simulink model "ball_impact"  (Simulink 8.1)
settings: Solver=ode4  SolverMode=SingleTasking  StartTime=0.0  StopTime=inf  FixedStep=0.0005  RelTol=1e-3
StartFcn:
  |  warndlg('Dexterit-E models cannot run under simulation. Please compile your model and run it from within Dexterit-E.');set_param(bdroot,'SimulationCommand','stop')
undefined symbols (not defined in the file or in its folder): CreateParameterTableGUI, slselsubs
libraries: xpclib x30, simulink x8, KINARM_general x3, KINARM_loads x2, Video x2, KINARM_EP_loads x1
(part 4 of 5)

== matlab function DataLogging/Poll KINARM/Create KINARM Data Array ==
  settings: fimath=|
      | fimath(...
      | 'RoundMode', 'floor',...
      | 'OverflowMode', 'wrap',...
      | 'ProductMode', 'KeepLSB', 'ProductWordLength', 32,...
      | 'SumMode', 'KeepLSB', 'SumWordLength', 32,...
      | 'CastBeforeSum', false)
  data: robot_calibrations input double; robot_hardware_settings input double; force_sensor_data input double; robot_data input double; servo_update_count input double; delay_estimates input double; primary_encoder_data input double; ep_calibration_button_bitfield input double; torque_command input double; hand_feedback_settings input double; kinarm_data output double; dominant_arm input double; primary_encoder_data_out output double; gaze_data input double
% This function constructs a matrix of KINARM-related data called "KINdata". This matrix consists of three rows: the first two are each
% for data related to the respective robot (i.e. row 1 is for robot 1 data, row 2 for robot 2 data, etc.), and the third row is for data
% not specific to either arm. Each row of the matrix is currently of length 50, though not all elements in each row are used.
function [kinarm_data, primary_encoder_data_out]= create_KINARM_data_array(robot_calibrations, robot_hardware_settings, force_sensor_data, ...
                                                      robot_data, servo_update_count, delay_estimates, primary_encoder_data, ...
                                                      ep_calibration_button_bitfield, torque_command, hand_feedback_settings, dominant_arm, gaze_data)

kinarm_data = zeros(3,50);
primary_encoder_data_out = zeros(2,6);

% Create the rows of robot-specific data. The utility function create_robot_row is used to assemble the values for each row. 
% The last section of that function (in which the row elements are assigned individually) documents the row contents.
kinarm_data(1,:) = create_robot_row(robot_calibrations(1:8), robot_hardware_settings(1:12), ...
                                    force_sensor_data(1:7), robot_data(1:10), torque_command(1:2));

kinarm_data(2,:) = create_robot_row(robot_calibrations(9:16), robot_hardware_settings(13:24), ...
                                    force_sensor_data(8:14), robot_data(11:20), torque_command(3:4));
								
% Create the last row of KINdata, which contains information not specific to any single arm.
kinarm_data(3,1) = dominant_arm;                     % dominant KINARM for the experiment (1: arm 1, 2: arm 2)
kinarm_data(3,2) = hand_feedback_settings(5);        % duration of feed forward for position of hand feedback (s)
kinarm_data(3,3) = hand_feedback_settings(1);        % hand feedback arm (0: none, 1: dominant, 2: non-dominant, 3: both, 4: controlled by task program)
kinarm_data(3,4) = hand_feedback_settings(2);        % hand feedback settings source (0: GUI, 1: from task program)
kinarm_data(3,5) = hand_feedback_settings(4);        % feedback colour (RRRGGGBBB string converted to integer)
kinarm_data(3,6) = hand_feedback_settings(3);        % feedback radius (m)
kinarm_data(3,7) = 1;                                % global load enable set by BKIN client software (no longer an option; thus always on)
kinarm_data(3,8) = delay_estimates(1);               % primary encoders velocity delay estimate (s)
kinarm_data(3,9) = delay_estimates(2);               % primary encoders acceleration delay estimate (s)
kinarm_data(3,10) = delay_estimates(3);              % secondary encoders velocity delay estimate (s)
kinarm_data(3,11) = delay_estimates(4);              % secondary encoders acceleration delay estimate (s)
kinarm_data(3,12) = servo_update_count;              % servo update count
kinarm_data(3,13) = ep_calibration_button_bitfield;  % EP calibration button status bitfield

gaze_available = gaze_data(1);
kinarm_data(3,14) = gaze_available;              % is Gaze tracking hardware available
kinarm_data(3,15) = hand_feedback_settings(6);   % Gaze feedback (0: on, 1: controlled by task program)

if gaze_available
    kinarm_data(3,16) = gaze_data(2);            % Gaze X location in global coordinates
    kinarm_data(3,17) = gaze_data(3);            % Gaze Y location in global coordinates
    kinarm_data(3,18) = gaze_data(4);            % Gaze Timestamp in seconds
    kinarm_data(3,19) = gaze_data(5);            % Gaze pupil area
    kinarm_data(3,20) = gaze_data(6);          % Gaze Event ID
    kinarm_data(3,21) = gaze_data(7);          % Gaze Event start time in seconds
    kinarm_data(3,22) = gaze_data(8);          % Gaze Event end time in seconds    
else
    kinarm_data(3,16) = -100;                    % Gaze X location in global coordinates
    kinarm_data(3,17) = -100;                    % Gaze Y location in global coordinates
    kinarm_data(3,18) = -100;                    % Gaze Timestamp in seconds
    kinarm_data(3,19) = -100;                    % Gaze Timestamp in seconds
end

% Create the two rows of primary encoder data. These outputs are analogous to the L1/L2 outputs in kinarm_data, the difference being that
% these are always derived from the primary encoders while the contents of kinarm_data is derived from the primary or secondary encoders
% (depending on the user's choice of whether or not to use the secondary encoders in the GUI).
for i = 1:2
	offset = (i-1)*6;
    
    relative_shoulder_angle = primary_encoder_data(1 + offset);
    relative_elbow_angle = primary_encoder_data(2 + offset);
    shoulder_velocity = primary_encoder_data(3 + offset);
    elbow_velocity = primary_encoder_data(4 + offset);
    shoulder_acceleration = primary_encoder_data(5 + offset);
    elbow_acceleration = primary_encoder_data(6 + offset);

    shoulder_angle_offset = robot_calibrations(1 + (i-1)*8);
    elbow_angle_offset = robot_calibrations(2 + (i-1)*8);
	L1 = robot_calibrations(5 + (i-1)*8);                               % L1 (upper arm segment) length (m)
	L3_error = robot_calibrations(8 + (i-1)*8);                         % L3 error, the difference between lengths L3 and L5 (m)
    
    hwoffset = (i-1)*12;
	robot_orientation = robot_hardware_settings(7 + hwoffset);          % robot orientation (1: right-handed from robot perspective, -1: left-handed from robot perspective)
 	L5 = robot_hardware_settings(3 + hwoffset);                         % L5 segment length (m)
	L2_L5_angle = robot_hardware_settings(4 + hwoffset);                % angle of L2 relative to L5 (rad)
    robot_type = robot_hardware_settings(1 + hwoffset);
    isExo = robot_type == 0 || robot_type == 2;
    
	% Before proceeding, the shoulder and elbow angles are shifted by the offsets determined by the calibration. If the calibration has been
	% performed correctly, this ensures that the angle of 0 corresponds to when the arm is aligned with the coronal plane. In the case of the 
	% elbow angle for a KINARM EXO, an extra correction is performed (using a utility function, and according to the current calibration) to 
	% account for small imperfections in the parallelogram of KINARM links caused by differences in the lengths of L3 and L5 (which are 
	% theoretically equal).
	shoulder_angle = relative_shoulder_angle + shoulder_angle_offset;

	% If the robot is an Exoskeleton, use the correct_elbow_angle function to account for imperfections on the KINARM robot parallelogram structure
	if isExo  
		[angle_corr, vel_corr, acc_corr] = correct_elbow_angle(relative_elbow_angle + elbow_angle_offset, elbow_velocity, elbow_acceleration, L2_L5_angle, L1, L5, L3_error);				
		elbow_angle = relative_elbow_angle + elbow_angle_offset + angle_corr;
		elbow_velocity = elbow_velocity + vel_corr;
		elbow_acceleration = elbow_acceleration + acc_corr;		
	else
		elbow_angle = relative_elbow_angle + elbow_angle_offset;
	end

    L1_angle = shoulder_angle;
    L2_angle = shoulder_angle + elbow_angle;

    L1_velocity = shoulder_velocity;
    L2_velocity = shoulder_velocity + elbow_velocity;

    L1_acceleration = shoulder_acceleration;
    L2_acceleration = shoulder_acceleration + elbow_acceleration;

	% a robot_orientation < 0 means that the robot is left-handed from its perspective (i.e. if you look at the robot structure, 
	% and pretend that it is a humanoid, the robot itself looks left-handed).  For an Exoskeleton robot, this is the
	% robot that the left-hand of the subject grabs. For an EP robot, this is the robot that the subjec'ts right-hand grabs.  
	
    if robot_orientation < 0
        L1_angle = -L1_angle + pi;
        L2_angle = -L2_angle + pi;

        L1_velocity = -L1_velocity;
        L2_velocity = -L2_velocity;

        L1_acceleration = -L1_acceleration;
        L2_acceleration = -L2_acceleration;
    end

    primary_encoder_data_out(i,1) = L1_angle;
    primary_encoder_data_out(i,2) = L2_angle;
    
    primary_encoder_data_out(i,3) = L1_velocity;
    primary_encoder_data_out(i,4) = L2_velocity;
    
    primary_encoder_data_out(i,5) = L1_acceleration;
    primary_encoder_data_out(i,6) = L2_acceleration;
end


%%%%%%%%%%%%%%%%%%%%%%%%%%%%%%%%%%%%%%%%%%%%%%%%%%%%%%%%%%%%%%%%%%%%%%%%%%%%%%%%%%%%%%%%%%%%%%%%%%%%%%%%%%%%%%%%%%%%%%%%
%%%%%%%%%%%%%%%%%%%%%%%%%%%%%%%%%%%%%%%%%%%%%%%%%%%%%%%%%%%%%%%%%%%%%%%%%%%%%%%%%%%%%%%%%%%%%%%%%%%%%%%%%%%%%%%%%%%%%%%%
% This function creates a row of arm-specific data for the KINARM data matrix. 
function robot_row = create_robot_row(calibration, hardware_settings, force_sensor_data, robot_data, torque_command)

% Extract the relevant information from each input array.
shoulder_angle_offset = calibration(1);            % offset added to motion control card shoulder angle to get real angle (rad)
elbow_angle_offset = calibration(2);               % offset added to motion control card elbow angle to get real angle (rad)
shoulder_position_x = calibration(3);              % shoulder x position (m) (global coordinates)
shoulder_position_y = calibration(4);              % shoulder y position (m) (global coordinates)
L1 = calibration(5);                               % L1 (upper arm segment) length (m)
L2 = calibration(6);                               % L2 (forearm segment) length (m); segment length puts distal end in line with subject pointer
pointer_offset = calibration(7);                   % perpendicular distance from L2 to subject pointer (m)
L3_error = calibration(8);                         % L3 error, the difference between lengths L3 and L5 (m)

robot_type = hardware_settings(1);                 % robot type (0: EXO, 1: EP, 2:NHP)
isExo = robot_type == 0 || robot_type == 2;
isEP = robot_type == 1;
L5 = hardware_settings(3);                         % L5 segment length (m)
L2_L5_angle = hardware_settings(4);                % angle of L2 relative to L5 (rad)
force_sensor_angle_offset = hardware_settings(5);  % offset of force sensor from forearm linkage (rad)
robot_orientation = hardware_settings(7);          % robot orientation (1: right-handed from robot perspective, -1: left-handed from robot perspective)

force_sensor_force_u = force_sensor_data(1);       % force sensor u force (N)
force_sensor_force_v = force_sensor_data(2);       % force sensor v force (N)
force_sensor_force_w = force_sensor_data(3);       % force sensor w force (N)
force_sensor_torque_u = force_sensor_data(4);      % force sensor u torque (Nm) 
force_sensor_torque_v = force_sensor_data(5);      % force sensor v torque (Nm)
force_sensor_torque_w = force_sensor_data(6);      % force sensor w torque (Nm)
force_sensor_timestamp = force_sensor_data(7);      % force sensor w torque (Nm)

relative_shoulder_angle = robot_data(1);        % current shoulder joint angle (rad)
relative_elbow_angle = robot_data(2);           % current elbow joint angle (rad)
shoulder_velocity = robot_data(3);                 % shoulder joint angular velocity (rad/s)
elbow_velocity = robot_data(4);                    % elbow joint angular velocity (rad/s)
shoulder_acceleration = robot_data(5);             % shoulder joint angular acceleration (rad/s^2)
elbow_acceleration = robot_data(6);                % elbow joint angular acceleration (rad/s^2)
filtered_shoulder_velocity = robot_data(7);        % filtered shoulder velocity (rad/s)
filtered_elbow_velocity = robot_data(8);           % filtered elbow velocity (rad/s)
motor1_status = robot_data(9);                     % motor 1 status
motor2_status = robot_data(10);                    % motor 2 status

shoulder_torque_cmd = torque_command(1);	       % commanded shoulder torque (Nm)
elbow_torque_cmd = torque_command(2);              % commanded elbow torque (Nm)



% With the inputs unpacked, start using them to compute other values that will be included in the data array. Some inputs are included in the
% array directly, but the kinematic data is also developed from the joint-based information supplied by the polling function into information 
% about the arm segments, the elbow, and the hand/fingertip as described in the following sections.

% Before proceeding, the shoulder and elbow angles are shifted by the offsets determined by the calibration. If the calibration has been
% performed correctly, this ensures that the angle of 0 corresponds to when the arm is aligned with the coronal plane. In the case of the 
% elbow angle for a KINARM EXO, an extra correction is performed (using a utility function, and according to the current calibration) to 
% account for small imperfections in the parallelogram of KINARM links caused by differences in the lengths of L3 and L5 (which are 
% theoretically equal).
shoulder_angle = relative_shoulder_angle + shoulder_angle_offset;

% If the robot is an Exoskeleton, use the correct_elbow_angle function to account for imperfections on the KINARM robot parallelogram structure
if isExo
	[angle_corr, vel_corr, acc_corr] = correct_elbow_angle(relative_elbow_angle + elbow_angle_offset, elbow_velocity, elbow_acceleration, L2_L5_angle, L1, L5, L3_error);
	elbow_angle = relative_elbow_angle + elbow_angle_offset + angle_corr;
	elbow_velocity = elbow_velocity + vel_corr;
	elbow_acceleration = elbow_acceleration + acc_corr;
else
	elbow_angle = relative_elbow_angle + elbow_angle_offset;
end

% Convert robot orientation as supplied in the hardware settings (a scaling factor used to calculate robot data) to the number 1 or 2,
% indicating which of the subject's arms will normally be using the robot: right or left, respectively. This is done to be consistent 
% with previous versions of the TDK. Note that the robot orientations of KINARM EP robots are "opposite" those for KINARM EXOs when.
if (isEP && robot_orientation < 0.0) || (isExo && robot_orientation > 0.0)
    arm_orientation = 1;  % right arm orientation expected for subject
else
    arm_orientation = 2;  % left arm orientation expected for subject
end

% Create a motor status variable for the robot that is consistent with previous versions of the TDK: the value forms a bitfield in
% which non-zero bits indicate a motor is disabled or faulted. The least significant bit is motor 1; the next is motor 2.
motor_status = motor2_status * 2 + motor1_status;

% Calculate segment information, i.e. positions, velocities, and accelerations for L1 and L2. "Segment-based" values here differ from the
% "joint-based" values in a few ways, though they are still expressed in angles:
%   i) elbow angles are no longer shoulder-relative (that is, L2 angles are not relative to L1)
%  ii) positions are expressed with the corrections calculated above
% iii) all angles are expressed in the same system, where 0 is the angular position of the exoskeleton right arm when aligned with the 
%      coronal plane and positive changes in angle correspond to counterclockwise movements.
%
% This section also determines the torque commands for motor 1 (shoulder) and motor 2 (elbow). When a positive torque is applied to the 
% forearm linkage by motor 2 it causes the same positive force on the upper arm linkage, so the torque applied to motor 1 is the desired
% shoulder torque less any torque commanded at the elbow.

L1_angle = shoulder_angle;
L2_angle = shoulder_angle + elbow_angle;

pointer_angle = shoulder_angle + elbow_angle + pi/2;
    
L1_velocity = shoulder_velocity;
L2_velocity = shoulder_velocity + elbow_velocity;
	
L1_acceleration = shoulder_acceleration;
L2_acceleration = shoulder_acceleration + elbow_acceleration;
    
M1_torque_cmd = shoulder_torque_cmd - elbow_torque_cmd;
M2_torque_cmd = elbow_torque_cmd;

% a robot_orientation < 0 means that the robot is left-handed from its perspective (i.e. if you look at the robot structure, 
% and pretend that it is a humanoid, the robot itself looks left-handed).  For an Exoskeleton robot, this is the
% robot that the left-hand of the subject grabs. For an EP robot, this is the robot that the subjec'ts right-hand grabs.  

if (robot_orientation == -1)
    L1_angle = -L1_angle + pi;
    L2_angle = -L2_angle + pi;
    
    pointer_angle = -pointer_angle + pi;
    
    L1_velocity = -L1_velocity;
    L2_velocity = -L2_velocity;
    
    L1_acceleration = -L1_acceleration;
    L2_acceleration = -L2_acceleration;
    
    M1_torque_cmd = -M1_torque_cmd;
    M2_torque_cmd = -M2_torque_cmd;
end

% Calculate elbow information, i.e. position, velocity, and acceleration, in X-Y space rather than joint angles.
elbow_position_x = shoulder_position_x + (L1 * cos(L1_angle));
elbow_position_y = shoulder_position_y + (L1 * sin(L1_angle));

elbow_velocity_x = -L1 * sin(L1_angle) * L1_velocity;
elbow_velocity_y =  L1 * cos(L1_angle) * L1_velocity;

elbow_acceleration_x = -L1 * (( cos(L1_angle) * L1_velocity^2) + (sin(L1_angle) * L1_acceleration));
elbow_acceleration_y =  L1 * ((-sin(L1_angle) * L1_velocity^2) + (cos(L1_angle) * L1_acceleration));

% Calculate fingertip/subject pointer/hand feedback information, i.e. position, velocity, and acceleration, in X-Y space.
hand_position_x = elbow_position_x + (L2 * cos(L2_angle)) + (pointer_offset * cos(pointer_angle));
hand_position_y = elbow_position_y + (L2 * sin(L2_angle)) + (pointer_offset * sin(pointer_angle));

hand_velocity_x = elbow_velocity_x - (L2 * sin(L2_angle) * L2_velocity) - (pointer_offset * sin(pointer_angle) * L2_velocity);
hand_velocity_y = elbow_velocity_y + (L2 * cos(L2_angle) * L2_velocity) + (pointer_offset * cos(pointer_angle) * L2_velocity);

hand_acceleration_x = elbow_acceleration_x - (L2 * (( cos(L2_angle) * L2_velocity^2) + (sin(L2_angle) * L2_acceleration))) - ...
    (pointer_offset * (( cos(pointer_angle) * L2_velocity^2) + (sin(pointer_angle) * L2_acceleration)));
hand_acceleration_y = elbow_acceleration_y + (L2 * ((-sin(L2_angle) * L2_velocity^2) + (cos(L2_angle) * L2_acceleration))) + ...
    (pointer_offset * ((-sin(pointer_angle) * L2_velocity^2) + (cos(pointer_angle) * L2_acceleration)));

% Calculate force sensor data for EP robots, or zero it for EXO robots. On each EP robot the force sensor is mounted at known angle to 
% the forearm linkage, which is specified as an input to this block. Two variants of the data are calculated: i) scaled in the force 
% sensor's local coordinate system ("uvw"), and ii) transformed to be in the global coordinate system ("xyz").
if isEP
    
    force_sensor_force_u = force_sensor_force_u / 1000000.0;  % scale values to SI using factors defined in force sensor configurations
    force_sensor_force_v = force_sensor_force_v / 1000000.0;
    force_sensor_force_w = force_sensor_force_w / 1000000.0;

    force_sensor_torque_u = force_sensor_torque_u / 1000000.0;
    force_sensor_torque_v = force_sensor_torque_v / 1000000.0;
    force_sensor_torque_w = force_sensor_torque_w / 1000000.0;

    sensor_u_angle = L2_angle - force_sensor_angle_offset;
    sensor_v_angle = L2_angle - force_sensor_angle_offset - pi/2;
    
    force_sensor_force_x = force_sensor_force_u * cos(sensor_u_angle) + force_sensor_force_v * cos(sensor_v_angle);
    force_sensor_force_y = force_sensor_force_u * sin(sensor_u_angle) + force_sensor_force_v * sin(sensor_v_angle);
    force_sensor_force_z = -force_sensor_force_w;

    force_sensor_torque_x = double(force_sensor_torque_u * cos(sensor_u_angle) + force_sensor_torque_v * cos(sensor_v_angle));
    force_sensor_torque_y = double(force_sensor_torque_u * sin(sensor_u_angle) + force_sensor_torque_v * sin(sensor_v_angle));
    force_sensor_torque_z = double(-force_sensor_torque_w);
    
else
    force_sensor_force_u = 0.0;
    force_sensor_force_v = 0.0;
    force_sensor_force_w = 0.0;

    force_sensor_torque_u = 0.0;
    force_sensor_torque_v = 0.0;
    force_sensor_torque_w = 0.0;

    force_sensor_force_x = 0.0;
    force_sensor_force_y = 0.0;
    force_sensor_force_z = 0.0;

    force_sensor_torque_x = 0.0;
    force_sensor_torque_y = 0.0;
    force_sensor_torque_z = 0.0;
end

% Construct the arm data array. Its construction is laid out here explicitly to provide comments for each entry (some are repeats from above). 
robot_row = zeros(1,50);

robot_row(1,1) = L1;                            % L1 (upper arm segment) length (m)
robot_row(1,2) = L2;                            % L2 (forearm segment) length (m); segment length puts distal end in line with subject pointer
robot_row(1,3) = pointer_offset;                % perpendicular distance from L2 to subject pointer (m)
robot_row(1,4) = shoulder_position_x;           % shoulder x position (m) (global coordinates)
robot_row(1,5) = shoulder_position_y;           % shoulder y position (m) (global coordinates)
robot_row(1,6) = arm_orientation;               % subject's expected arm orientation (1: right, 2: left)
robot_row(1,7) = shoulder_angle;				% shoulder joint angle, with correction for offsets (see above) (rad)
robot_row(1,8) = elbow_angle;					% elbow joint angle, with correction for offsets (see above) (rad)
robot_row(1,9) = shoulder_velocity;             % shoulder joint angular velocity (rad/s)
robot_row(1,10) = elbow_velocity;               % elbow joint angular velocity (rad/s)
robot_row(1,11) = shoulder_acceleration;        % shoulder joint angular acceleration (rad/s^2)
robot_row(1,12) = elbow_acceleration;           % elbow joint angular acceleration (rad/s^2)
robot_row(1,13) = shoulder_torque_cmd;          % commanded shoulder torque (Nm)
robot_row(1,14) = elbow_torque_cmd;             % commanded elbow torque (Nm)
robot_row(1,15) = M1_torque_cmd;                % commanded motor 1 torque (shoulder torque less elbow torque) (Nm)
robot_row(1,16) = M2_torque_cmd;                % commanded motor 2 torque (Nm)
robot_row(1,17) = L1_angle;                     % upper arm angle with corrections, orientation-independent (see above) (rad)
robot_row(1,18) = L2_angle;                     % forearm angle with corrections, orientation and shoulder-independent (see above) (rad)
robot_row(1,19) = L1_velocity;                  % upper arm angular velocity, orientation-independent (see above) (rad/s)
robot_row(1,20) = L2_velocity;                  % forearm angular velocity, orientation and shoulder-independent (see above) (rad/s)
robot_row(1,21) = L1_acceleration;              % upper arm angular acceleration, orientation-independent (see above) (rad/s^2)
robot_row(1,22) = L2_acceleration;              % forearm angular acceleration, orientation and shoulder-independent (see above) (rad/s^2)
robot_row(1,23) = hand_position_x;              % fingertip position in x (m)
robot_row(1,24) = hand_position_y;              % fingertip position in y (m)
robot_row(1,25) = hand_velocity_x;              % fingertip velocity in x (m/s)
robot_row(1,26) = hand_velocity_y;              % fingertip velocity in y (m/s)
robot_row(1,27) = hand_acceleration_x;          % fingertip acceleration in x (m/s^2)
robot_row(1,28) = hand_acceleration_y;          % fingertip acceleration in y (m/s^2)
robot_row(1,29) = elbow_position_x;             % elbow position in x (m)
robot_row(1,30) = elbow_position_y;             % elbow position in y (m)
robot_row(1,31) = elbow_velocity_x;             % elbow velocity in x (m/s)
robot_row(1,32) = elbow_velocity_y;             % elbow velocity in y (m/s)
robot_row(1,33) = elbow_acceleration_x;         % elbow acceleration in x (m/s^2)
robot_row(1,34) = elbow_acceleration_y;         % elbow acceleration in y (m/s^2)
robot_row(1,35) = filtered_shoulder_velocity;   % filtered shoulder velocity from motion control card (rad/s)
robot_row(1,36) = filtered_elbow_velocity;      % filtered elbow velocity from motion control card (rad/s)
robot_row(1,37) = motor_status;                 % motor status (bitfield; each 0: motor enabled, 1: motor disabled/faulted)
robot_row(1,38) = force_sensor_force_u;         % force measured by force sensor along u in its local coordinate system (N)
robot_row(1,39) = force_sensor_force_v;         % force measured by force sensor along v in its local coordinate system (N)
robot_row(1,40) = force_sensor_force_w;         % force measured by force sensor along w in its local coordinate system (N)
robot_row(1,41) = force_sensor_torque_u;        % torque measured by force sensor along u in its local coordinate system (Nm)
robot_row(1,42) = force_sensor_torque_v;        % torque measured by force sensor along v in its local coordinate system (Nm)
robot_row(1,43) = force_sensor_torque_w;        % torque measured by force sensor along w in its local coordinate system (Nm)
robot_row(1,44) = force_sensor_force_x;         % force measured by force sensor along x in the global coordinate system (N)
robot_row(1,45) = force_sensor_force_y;         % force measured by force sensor along y in its local coordinate system (N)
robot_row(1,46) = force_sensor_force_z;         % force measured by force sensor along z in its local coordinate system (N)
robot_row(1,47) = force_sensor_torque_x;        % torque measured by force sensor along x in its local coordinate system (Nm)
robot_row(1,48) = force_sensor_torque_y;        % torque measured by force sensor along y in its local coordinate system (Nm)
robot_row(1,49) = force_sensor_torque_z;        % torque measured by force sensor along z in its local coordinate system (Nm)
robot_row(1,50) = force_sensor_timestamp;       % The timestamp from the force sensor(s)



function [angle_corr vel_corr acc_corr] = correct_elbow_angle(elbow_angle, elbow_vel, elbow_acc, theta2_5, L1, L5, L3_error)

% this function corrects for errors in non-perfect parallelogram structure
% It assumes that L5 is exact (because it is machined from one
% piece of material) and that there is an error in L3.  Note: although
% there could also be an error in L4, this 'correction' factor can
% effectively account for both errors by computing an equivalent L3_error

L3 = L5 + L3_error;

theta1_3 = theta2_5 - elbow_angle;		%actual angle between links 1 and 3
dtheta1_3dt = - elbow_vel;
d2theta1_3d2t = - elbow_acc;

% The following shifts theta1_3 to between -pi and pi and stores the shift.
% Although theta1_3 should always be between 0 and pi, during initial
% calibration there might be some values outside of that range.
theta1_3_2pi_offset = floor( (theta1_3 + pi)/(2 *pi) );
theta1_3 = theta1_3 - theta1_3_2pi_offset * 2 * pi;

%Option 1a
a = 4 * L3 * L5 - 4*L1*L5*cos(theta1_3);
b = -4 * L1 * L5 * sin(theta1_3);
c = L3^2 + L5^2 - 2 * L3 * L5 - 2 * L1 * L3_error * cos(theta1_3) ;

dbdt = -4 * L1 * L5 * cos(theta1_3) * dtheta1_3dt;
dcdt = 2 * L1 * L3_error * sin(theta1_3) * dtheta1_3dt;

d2bdt2 = 4 * L1 * L5 * sin(theta1_3) * dtheta1_3dt^2 -4 * L1 * L5 * cos(theta1_3) * d2theta1_3d2t;
d2cdt2 = 2 * L1 * L3_error * cos(theta1_3) * dtheta1_3dt^2 + 2 * L1 * L3_error * sin(theta1_3) * d2theta1_3d2t;

sqroot = sqrt( b^2 - 4 * a * c);

if sqroot > 0
	if b > 0
		sinU = (-b + sqroot ) / (2 * a);
		dsinUdt = (-dbdt + 1/2 * 1/sqroot * (2*b*dbdt -4*a*dcdt) ) / (2 * a);
		d2sinUdt2 = (-d2bdt2 - 1/4 * 1/sqroot^3 * (2*b*dbdt -4*a*dcdt)^2 + 1/2 * 1/sqroot * (2*dbdt^2 + 2*b*d2bdt2 -4*a*d2cdt2) ) / (2 * a); 
	else
		sinU = (-b - sqroot ) / (2 * a);
		dsinUdt = (-dbdt - 1/2 * 1/sqroot * (2*b*dbdt -4*a*dcdt) ) / (2 * a);
		d2sinUdt2 = (-d2bdt2 + 1/4 * 1/sqroot^3 * (2*b*dbdt -4*a*dcdt)^2 - 1/2 * 1/sqroot * (2*dbdt^2 + 2*b*d2bdt2 -4*a*d2cdt2) ) / (2 * a); 
	end
else
	sinU = -b / (2 * a);
	dsinUdt = -dbdt / (2 * a);
	d2sinUdt2 = -d2bdt2 / (2 * a); 
end	

if sinU > 1
	sinU = 1;
elseif sinU < -1
	sinU = -1;
end

U = asin(sinU);

theta1_5_corr = 2 * U;
vel1_5_corr = 2 / sqrt(1 - sinU^2) * dsinUdt;
acc1_5_corr = 2 / (1 - sinU^2)^(3/2) * sinU * (dsinUdt)^2 + 2 / sqrt(1 - sinU^2) * d2sinUdt2;

angle_corr = - theta1_5_corr;
vel_corr = - vel1_5_corr;
acc_corr = - acc1_5_corr;

== matlab function GUI Control/Run Command Subsystem/Embedded MATLAB Function ==
  data: x input double; y output double; z output double
function [y,z]= fcn(x)
% This block determines the run_command input of the task execution control
% subsystem (y), as well as the value of the task control button Goto (z).

persistent u
persistent v

if isempty(u)
    u = 0;
end

if isempty(v)
    v = 0;
end

% To the run_command input, only output a 1 or a 0 ('run' or 'pause')
% according to the last received status for the Go/Pause button.
if x < 2 && u ~= x
    u = x;
end

y = u;

% To the Goto block, only output a non-zero value on the first receipt of 
% a block index > 1 (i.e. not the Go/Pause button).
if x > 1 && x ~= v
    v = x;
    if v == 255
        z = 0;
    else     
        z = v;
    end
else
    z = 0;
end

== stateflow chart GUI Control/Task Execution Control Subsystem/Task Execution Control Machine ==
  settings: sampleTime=0.0005
  state PausedBetweenTrials/
    task_status = 3;
  state Finished/
    task_status = 4;
  state PausedBetweenBlocks/
    task_status = 3;
  state InTrial/
    trial_in_set++;
    trial_in_block++;
    trial_in_mini_block++;
    tp  = trial_queue[trial_in_mini_block];
    state Running/
      task_status = 2;
    state SkipTrial/
      e_exit_trial;
    state Paused/
      task_status = 3;
    state RepeatTrialLater/
      e_exit_trial;
    state RepeatTrialNow/
      trial_in_mini_block--;
      e_exit_trial;
    (junction 209) -> SkipTrial [order 1] : [pause_type == 1]
    (junction 210) -> RepeatTrialNow [order 1] : [pause_type == 2]
    (junction 211) -> RepeatTrialLater [order 1] : [pause_type == 3]
    (default) -> Running
    Running -> (junction 209) : [run_command <> 1 && pause_type > 0]
    (junction 209) -> (junction 210) [order 2]
    (junction 210) -> (junction 211) [order 2]
    (junction 211) -> (junction 212) [order 2]
    Paused -> Running : [run_command == 1]
    (junction 212) -> Paused
  state Ready/
    task_status = 1;
    tp = 0;
    block = 0;
    trial_in_block = 0;
    block_in_set = 0;
    trial_in_set = 0;
    trial_in_mini_block = 0;
  (default) -> Ready
  (junction 253) -> Finished [order 2] : // Finish if using a task program-specified block sequence
      | // and the block index input from the program is invalid.
      | [use_task_protocol_block_sequence_flag == 0 && ...
      |  (next_task_program_specified_block == 0 || ...
      |   next_task_program_specified_block > max_block_definitions)]
  (junction 257) -> Finished [order 1] : // Finish if using a task protocol block sequence
      | // and that sequence has finished.
      | [i == task_protocol_block_sequence_length && temp <= block_in_set]
  Ready -> (junction 251) : [run_command == 1]
      | { srand(seed); }
  (junction 251) -> (junction 252)
  (junction 252) -> (junction 253)
  (junction 253) -> (junction 254) [order 1] : // If specified, use task protocol block sequence.
      | [use_task_protocol_block_sequence_flag == 1]
      | {
      | i = 1;
      | temp = task_protocol_block_sequence[1][2];
      | }
  (junction 256) -> (junction 254) [order 1] : [temp <= block_in_set && ...
      |  i < task_protocol_block_sequence_length]
      | {
      | i++;
      | temp = temp + task_protocol_block_sequence[i][2];
      | }
  PausedBetweenBlocks -> (junction 251) : [run_command == 1]
  (junction 255) -> (junction 252) [order 1] : [run_command == 1]
  (junction 253) -> (junction 258) [order 3] : // Make user-input block index the next block.
      | { block = next_task_program_specified_block; }
  (junction 254) -> (junction 256)
  (junction 255) -> PausedBetweenBlocks [order 2]
  (junction 263) -> (junction 255)
  (junction 256) -> (junction 257) [order 2]
  (junction 257) -> (junction 260) [order 2] : // Make next task protocol block index the next block.
      | { block = task_protocol_block_sequence[i][1]; }
  (junction 258) -> (junction 259)
  (junction 260) -> (junction 259)
  (junction 259) -> (junction 261) : { block_in_set++;
      |   i = 1; }
  (junction 262) -> (junction 261) [order 1] : // Copy the trial list from the block definitions to the trial queue.
      | [i <= trial_queue_max_length && block > 0 && block_definitions[block][i+1] != 0]
      | {
      | trial_queue[i] = block_definitions[block][i+1];
      | i++;
      | }
  (junction 261) -> (junction 262)
  (junction 262) -> (junction 264) [order 2] : { trial_queue_length = i-1; }
  (junction 264) -> (junction 263) [order 2]
  (junction 265) -> (junction 263) [order 2]
  (junction 264) -> (junction 266) [order 1] : [trial_queue_length > 0]
      | { trial_in_block = 0; }
  (junction 265) -> (junction 266) [order 1] : // If there are any trials to repeat, assign them to the
      | // trial queue instead of advancing to the next block.
      | [repeat_list_length > 0]
      | {
      | trial_queue = repeat_list;
      | trial_queue_length = repeat_list_length;
      | repeat_list = 0;
      | repeat_list_length = 0;
      | }
  (junction 273) -> (junction 265) [order 1] : [trial_in_mini_block >= trial_queue_length]
  (junction 266) -> (junction 267) : { trial_in_mini_block = 0; }
  (junction 267) -> (junction 268) [order 2]
  (junction 267) -> (junction 269) [order 1] : // Randomize the block if the definition specifies to do so.
      | [block_definitions[block][1] == 1]
      | { i = 1; }
  (junction 268) -> (junction 271)
  (junction 269) -> (junction 270)
  (junction 270) -> (junction 271) [order 2]
  (junction 270) -> (junction 269) [order 1] : // Perform list randomization "a la Knuth".
      | [i <= trial_queue_length]
      | {
      | swap_index = fmod(rand(), trial_queue_length) + 1;
      | temp = trial_queue[swap_index];
      | trial_queue[swap_index] = trial_queue[i];
      | trial_queue[i] = temp;
      | i++;
      | }
  (junction 271) -> (junction 278)
  (junction 274) -> PausedBetweenTrials [order 2]
  PausedBetweenTrials -> InTrial : [run_command == 1]
  (junction 277) -> PausedBetweenTrials
  (junction 272) -> (junction 273) : // Add the current trial to the repeat list.
      | {
      | repeat_list_length++;
      | repeat_list[repeat_list_length] = tp;
      | }
  (junction 273) -> (junction 274) [order 2]
  (junction 275) -> (junction 272)
  (junction 276) -> (junction 273) [order 2]
  (junction 274) -> InTrial [order 1] : [run_command == 1]
  (junction 276) -> (junction 275) [order 1] : // Also add the current trial to the repeat list
      | // if the repeat trial flag is set and the task is
      | // running (either normally or until pausing at
      | // the next trial).
      | [repeat_trial_flag > 0 && ...
      |  (run_command == 1 || pause_type == 0)]
  (junction 279) -> (junction 275)
  (junction 280) -> (junction 276) [order 2]
  (junction 278) -> (junction 277) [order 1] : [run_command <> 1]
  (junction 278) -> InTrial [order 2]
  (junction 280) -> (junction 279) [order 1] : // Add the current trial to the repeat list if the
      | // task is paused and the selected pause type
      | // is to repeat the trial later, i.e. at the end of
      | // the block. This occurs independent of the
      | // repeat trial flag.
      | [run_command <> 1 && pause_type == 3]
  InTrial -> (junction 280) : e_trial_over
  data: repeat_trial_flag input double; task_status output uint32; tp output uint32; block output uint32; trial_in_block output uint32; block_in_set output uint32; trial_in_set output uint32; trial_queue local double size=499; repeat_list local double size=499; run_command input uint8; pause_type input double; seed input double; block_definitions input double; max_block_definitions input uint32; trial_queue_max_length input uint32 =499; use_task_protocol_block_sequence_flag input double; task_protocol_block_sequence input double; task_protocol_block_sequence_length input uint32; repeat_list_length local uint32; i local uint32 =1; swap_index local uint32; temp local uint32; next_task_program_specified_block input double; trial_queue_length local uint32 =499; trial_in_mini_block local uint32
  data block_definitions settings: description=|
      | Describes the set in terms of a sequence of blocks
      | Row 1 = Block 1
      | cols:
      | 1 = TL start_index (>=1)
      | 2 = TL end_index (>=1)
      | 3 = randomized (1/0)
      | 4 = reps ( > 0 )
  data task_protocol_block_sequence settings: description=|
      | Describes the set in terms of a sequence of blocks
      | Row 1 = Block 1
      | cols:
      | 1 = TL start_index (>=1)
      | 2 = TL end_index (>=1)
      | 3 = randomized (1/0)
      | 4 = reps ( > 0 )
  data task_protocol_block_sequence_length settings: description=|
      | Describes the set in terms of a sequence of blocks
      | Row 1 = Block 1
      | cols:
      | 1 = TL start_index (>=1)
      | 2 = TL end_index (>=1)
      | 3 = randomized (1/0)
      | 4 = reps ( > 0 )
  events: e_clk input EITHER_EDGE_EVENT; e_trial_over input EITHER_EDGE_EVENT; e_exit_trial output EITHER_EDGE_EVENT

== matlab function DataLogging/Poll KINARM/Force Sensor Control Subsystem/Force Sensor 1 Subsystem/Create timestamp ==
  data: times_in input double; timestamp_out output double
function timestamp_out = fcn(times_in)

persistent start_time
persistent last_time

if isempty(start_time)
   start_time = uint32(0);
end

if isempty(last_time)
    last_time = uint32(0);
end

if start_time == 0 && times_in(2) > 0
    start_time = times_in(2);
end

if times_in(2) < start_time
    start_time = -(last_time - start_time);
end

%F/T sensor clock runs at 7Khz according to the manual,
%using a 32 bit integer for this gives about 7 days before it will roll
%over. This means we need to account for roll overs in order to make
%analysis sane.
timestamp_out = double(times_in(2) - start_time) / 7000.0;
last_time = times_in(2);

== matlab function DataLogging/Poll KINARM/Force Sensor Control Subsystem/Force Sensor 2 Subsystem/Create timestamp ==
  data: times_in input double; timestamp_out output double
function timestamp_out = fcn(times_in)

persistent start_time
persistent last_time

if isempty(start_time)
   start_time = uint32(0);
end

if isempty(last_time)
    last_time = uint32(0);
end

if start_time == 0 && times_in(2) > 0
    start_time = times_in(2);
end

if times_in(2) < start_time
    start_time = -(last_time - start_time);
end

%F/T sensor clock runs at 7Khz according to the manual,
%using a 32 bit integer for this gives about 7 days before it will roll
%over. This means we need to account for roll overs in order to make
%analysis sane.
timestamp_out = double(times_in(2) - start_time) / 7000.0;
last_time = times_in(2);

== matlab function DataLogging/Poll KINARM/Monitor_status ==
  settings: fimath=|
      | fimath(...
      | 'RoundMode', 'floor',...
      | 'OverflowMode', 'wrap',...
      | 'ProductMode', 'KeepLSB', 'ProductWordLength', 32,...
      | 'SumMode', 'KeepLSB', 'SumWordLength', 32,...
      | 'CastBeforeSum', false)
  data: status_data input double; servo_counter input double; robotCount input double; force_scale output double; plcc_version input double
function force_scale = monitor_system_status(status_data, servo_counter, robotCount, plcc_version)

%This function must run at 1kHz so that the counter from the PMAC can be properly checked.
% i.e. this must run slower than the PMAC

persistent no_update_count;
persistent last_servo_counter;

if isempty(no_update_count)
   no_update_count = 0;
end

if isempty(last_servo_counter)
    last_servo_counter = uint32(0);
end

pmac_fault_state = uint32(status_data(2));
plcc_switch = status_data(3);
force_scale = 1;

%plcc versions >1000 are custom
if plcc_version >= 6.0 && plcc_version < 1000
    %if the task is running and the servo amp counter is not
    if plcc_switch == 4.0 && last_servo_counter == servo_counter
        no_update_count = no_update_count + 1;    
        %after 5 cycles with the counter not running we should kill forces.
        if no_update_count >= 5
            force_scale = 0;
        end
    else
        no_update_count = 0;
    end
    last_servo_counter = servo_counter; 
end

%plcc versions >1000 are custom
if plcc_version >= 7.0 && plcc_version < 1000
    %if it is unilateral and the robot state is faulted then kill the forces
    if robotCount == 1 && bitand(pmac_fault_state, 1) == 1
        force_scale = 0;
    %if the system is bilateral and either robot is faulted, kill forces.
    elseif robotCount == 2 && bitand(pmac_fault_state, 3) ~= 0
        force_scale = 0;
    end
end

if plcc_version == 0
    force_scale = 0;
end

== matlab function DataLogging/Receive_Gaze/Create timestamp ==
  data: time_in input double; timestamp_out output double; start_time_out output double
function [timestamp_out, start_time_out] = fcn(time_in)

persistent start_time
persistent last_time

if isempty(start_time)
   start_time = -1;
end

if isempty(last_time)
    last_time = -1;
end

if start_time == -1 && time_in ~= 0
    start_time = time_in;
end

%if the clock has flipped over then in order to get the time
%right this will add the time before the flip to the current time.
if time_in < start_time
    start_time = -(last_time - start_time);
end

timestamp_out = (time_in - start_time) / 1000.0;
last_time = time_in;
start_time_out = start_time;
